simulink model "AFC1_F_trainscg_15_15_15_controller_ep_1000_Nor_20250518"  (R2021a)
settings: Solver=VariableStepAuto  StartTime=0.0  StopTime=10.0  RelTol=1e-3
libraries: neural x50
(part 2 of 2)

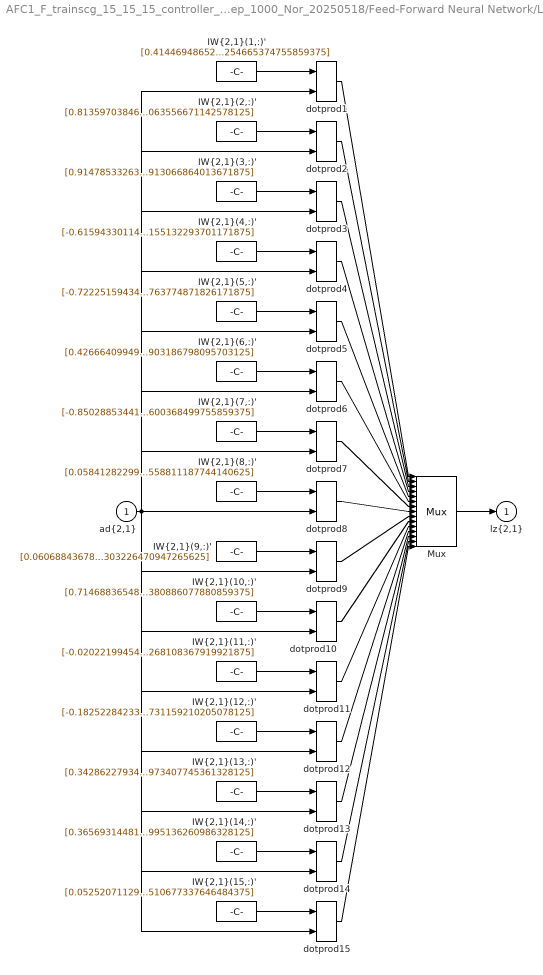
== system AFC1_F_trainscg_15_15_15_controller_ep_1000_Nor_20250518/Feed-Forward Neural Network/Layer 2/LW{2,1} ==
  "ad{2,1}" : Inport  PortDimensions=15
      mask Display: e = 0.06;c1 = [120 230 180]/255;c2 = ([120 230 180]+0)/(256+128);c3 = ([120 230 180]+128)/(256+128);patch([0 1 1 0],[0 0 1 1],c1);patch([0 1 1 1-e 1-e 0+e],[0 0 1 1-e 0+e 0+e],c2);patch([0 0 1 1-e 0+e 0+e],[0 1 1 1-e 1-e 0+e],c3);plot([0 1 1 0 0],[0 0 1 1 0]);
  "IW{2,1}(1,:)'" : Constant  Value=[0.414469486526158281680665140811470337212085723876953125;-0.2259536984836016670907810066637466661632061004638671875;-1.0195501104377717727089702748344279825687408447265625;0.54480850054258167514120714258751831948757171630859375;-0.1760777495828814431799713702275766991078853607177734375;0.5823251328806093862766601887415163218975067138671875;-0.54431412858791627940036050858907401561737060546875;0.5380581706717924017624454791075550019741058349609375;-0.9009348419158775822523921306128613650798797607421875;-0.7521354448038597428904949993011541664600372314453125;0.241917287870616615208518851432017982006072998046875;-0.84101322207548967480050805534119717776775360107421875;-0.64873063937154740177248868349124677479267120361328125;-0.60797567984407063779173086004448123276233673095703125;-0.659413490808771651785491485497914254665374755859375]
      mask Display: e = 0.06;c1 = [120 150 230]/255;c2 = ([120 150 230]+0)/383;c3 = ([120 150 230]+128)/383;patch([0 1 1 0],[0 0 1 1],c1);patch([0 1 1 1-e 1-e 0+e],[0 0 1 1-e 0+e 0+e],c2);patch([0 0 1 1-e 0+e 0+e],[0 1 1 1-e 1-e 0+e],c3);plot([0 1 1 0 0],[0 0 1 1 0]);disp('weights');
  "IW{2,1}(10,:)'" : Constant  Value=[0.7146883654878719571712508695782162249088287353515625;-0.08214663972938236746745843674943898804485797882080078125;0.55044775605694618025864883747999556362628936767578125;0.954649122831302765490590900299139320850372314453125;0.3557796049595560727851761839701794087886810302734375;0.77915393221201278972642967346473596990108489990234375;-0.8330343727947546739187600906006991863250732421875;-0.581189831958130564970588238793425261974334716796875;-0.4362662882391401542037101535242982208728790283203125;-0.588048968935513283184945976245217025279998779296875;0.968796624481943258189176049199886620044708251953125;0.712762216768441536629552501835860311985015869140625;-0.45158776578670067891607686760835349559783935546875;-0.050073148627536485932854048996887286193668842315673828125;-0.1291644265589745044220393310752115212380886077880859375]
      mask Display: e = 0.06;c1 = [120 150 230]/255;c2 = ([120 150 230]+0)/383;c3 = ([120 150 230]+128)/383;patch([0 1 1 0],[0 0 1 1],c1);patch([0 1 1 1-e 1-e 0+e],[0 0 1 1-e 0+e 0+e],c2);patch([0 0 1 1-e 0+e 0+e],[0 1 1 1-e 1-e 0+e],c3);plot([0 1 1 0 0],[0 0 1 1 0]);disp('weights');
  "IW{2,1}(11,:)'" : Constant  Value=[-0.020221994544841991048311768963685608468949794769287109375;0.39058790934535092542745360333356074988842010498046875;-0.267494483371077951261440830421634018421173095703125;0.008683861322354761991260119202706846408545970916748046875;-0.03148972773896197008269837169791571795940399169921875;0.2116872775745909651678999807700165547430515289306640625;0.25191957034316647678906520013697445392608642578125;0.1045826830775500315695580866304226219654083251953125;0.07719335609068078696282100281678140163421630859375;0.8958662425863372913426019295002333819866180419921875;0.7178776333677323595594543803599663078784942626953125;0.0823128711607351848389413362383493222296237945556640625;-0.1821172769517398759564485999362659640610218048095703125;0.784913646248323715326478122733533382415771484375;-1.033094077922761311327803923632018268108367919921875]
      mask Display: e = 0.06;c1 = [120 150 230]/255;c2 = ([120 150 230]+0)/383;c3 = ([120 150 230]+128)/383;patch([0 1 1 0],[0 0 1 1],c1);patch([0 1 1 1-e 1-e 0+e],[0 0 1 1-e 0+e 0+e],c2);patch([0 0 1 1-e 0+e 0+e],[0 1 1 1-e 1-e 0+e],c3);plot([0 1 1 0 0],[0 0 1 1 0]);disp('weights');
  "IW{2,1}(12,:)'" : Constant  Value=[-0.1825228423300189195543907771934755146503448486328125;-0.2116393226556184392617154799154377542436122894287109375;0.61085605728163583361123301074258051812648773193359375;0.7443810798191494715325688957818783819675445556640625;-0.62247861816263128087456379944342188537120819091796875;0.965093447760789313605300776544027030467987060546875;0.32188911589468460761054302565753459930419921875;0.25976677012884241690926501178182661533355712890625;0.390326078888663996480090645491145551204681396484375;-0.835857585804548275376646415679715573787689208984375;0.571117978530061076725132807041518390178680419921875;0.7300334446399059373788986704312264919281005859375;-0.06533126904650272959163004315996658988296985626220703125;-0.7992512801152766854784204042516648769378662109375;0.77556135590495778320274666839395649731159210205078125]
      mask Display: e = 0.06;c1 = [120 150 230]/255;c2 = ([120 150 230]+0)/383;c3 = ([120 150 230]+128)/383;patch([0 1 1 0],[0 0 1 1],c1);patch([0 1 1 1-e 1-e 0+e],[0 0 1 1-e 0+e 0+e],c2);patch([0 0 1 1-e 0+e 0+e],[0 1 1 1-e 1-e 0+e],c3);plot([0 1 1 0 0],[0 0 1 1 0]);disp('weights');
  "IW{2,1}(13,:)'" : Constant  Value=[0.342862279348052023664195075980387628078460693359375;0.366831733935956805225941934622824192047119140625;0.5101541980141670595827463330351747572422027587890625;0.1760521106169949945297048543579876422882080078125;-0.0099883500195583341252358877682127058506011962890625;0.0553601386768847181230057685752399265766143798828125;0.459503710634442175120284446165896952152252197265625;-0.9360179684748661799176261411048471927642822265625;-0.0017679730348210132007125139352865517139434814453125;-0.7885811468365571119676360467565245926380157470703125;0.0267548371751498148540804322692565619945526123046875;-0.3042416113454777804037121313740499317646026611328125;0.5279141569839131964414491449133493006229400634765625;0.4910921474034346534409678497468121349811553955078125;-0.606683617264736074758957329322583973407745361328125]
      mask Display: e = 0.06;c1 = [120 150 230]/255;c2 = ([120 150 230]+0)/383;c3 = ([120 150 230]+128)/383;patch([0 1 1 0],[0 0 1 1],c1);patch([0 1 1 1-e 1-e 0+e],[0 0 1 1-e 0+e 0+e],c2);patch([0 0 1 1-e 0+e 0+e],[0 1 1 1-e 1-e 0+e],c3);plot([0 1 1 0 0],[0 0 1 1 0]);disp('weights');
  "IW{2,1}(14,:)'" : Constant  Value=[0.36569314481354375789834421084378845989704132080078125;0.463132816817762360539489918664912693202495574951171875;-0.307263751603320367511429367368691600859165191650390625;-0.6367346347823830132739431064692325890064239501953125;-0.72715071881299753187022361089475452899932861328125;0.10794316621904233299833464343464584089815616607666015625;0.78150423265064450362160641816444694995880126953125;0.2294268382342810053131643144297413527965545654296875;0.071602111502226506445367704145610332489013671875;-0.7159177561920035959275310233351774513721466064453125;-0.644795078988269931841159632313065230846405029296875;-0.2246800037110795733585888456218526698648929595947265625;0.6264676586349986475710238664760254323482513427734375;0.491901981953333178321230434448807500302791595458984375;-0.8295669794164439725392412583460099995136260986328125]
      mask Display: e = 0.06;c1 = [120 150 230]/255;c2 = ([120 150 230]+0)/383;c3 = ([120 150 230]+128)/383;patch([0 1 1 0],[0 0 1 1],c1);patch([0 1 1 1-e 1-e 0+e],[0 0 1 1-e 0+e 0+e],c2);patch([0 0 1 1-e 0+e 0+e],[0 1 1 1-e 1-e 0+e],c3);plot([0 1 1 0 0],[0 0 1 1 0]);disp('weights');
  "IW{2,1}(15,:)'" : Constant  Value=[0.05252071129474260302583132897780160419642925262451171875;-0.1330683727143766870160135340483975596725940704345703125;-0.5847519347945955292544795156572945415973663330078125;-0.63886919009627873844436862782458774745464324951171875;-0.8971754527457538319623608913389034569263458251953125;0.54648741890165108969767970847897231578826904296875;0.964606445767212772324228353681974112987518310546875;-0.2751770754538946928136056158109568059444427490234375;-0.10963366940791541281896570581011474132537841796875;-0.667079118247158486809667010675184428691864013671875;-0.2028210065283138074931912342435680329799652099609375;-0.877611894985142360070540235028602182865142822265625;-0.79725683317359485879904923422145657241344451904296875;0.124435927059549644724256722838617861270904541015625;-0.416150764835760911264372907680808566510677337646484375]
      mask Display: e = 0.06;c1 = [120 150 230]/255;c2 = ([120 150 230]+0)/383;c3 = ([120 150 230]+128)/383;patch([0 1 1 0],[0 0 1 1],c1);patch([0 1 1 1-e 1-e 0+e],[0 0 1 1-e 0+e 0+e],c2);patch([0 0 1 1-e 0+e 0+e],[0 1 1 1-e 1-e 0+e],c3);plot([0 1 1 0 0],[0 0 1 1 0]);disp('weights');
  "IW{2,1}(2,:)'" : Constant  Value=[0.81359703846538866667259526366251520812511444091796875;-0.69557176260931818934096781958942301571369171142578125;-0.35735248624277360374179579594056122004985809326171875;0.94837000715828800867512882177834399044513702392578125;0.427155190796831452093584857720998115837574005126953125;0.2002273250899879730724251203355379402637481689453125;-0.003811417607220590753058786503970623016357421875;0.162892975750795532263737186440266668796539306640625;-0.0208600216453564968333012075163424015045166015625;-0.0192854130639636967003980316803790628910064697265625;0.147419529682396355241280616610310971736907958984375;-0.963420188137352528912060734000988304615020751953125;0.327449263835897175223266231114394031465053558349609375;-0.2810892969728204793256054472294636070728302001953125;0.189692708737160764531637369145755656063556671142578125]
      mask Display: e = 0.06;c1 = [120 150 230]/255;c2 = ([120 150 230]+0)/383;c3 = ([120 150 230]+128)/383;patch([0 1 1 0],[0 0 1 1],c1);patch([0 1 1 1-e 1-e 0+e],[0 0 1 1-e 0+e 0+e],c2);patch([0 0 1 1-e 0+e 0+e],[0 1 1 1-e 1-e 0+e],c3);plot([0 1 1 0 0],[0 0 1 1 0]);disp('weights');
  "IW{2,1}(3,:)'" : Constant  Value=[0.9147853326346122582179987148265354335308074951171875;0.063908989507247715433635448789573274552822113037109375;-0.14686911338523411796330719880643300712108612060546875;-0.3143718417331886616494784902897663414478302001953125;0.6604950288199826768931188780697993934154510498046875;0.8262060339228549654677635771804489195346832275390625;0.801704977064009671750000052270479500293731689453125;0.856626124628375951175485170097090303897857666015625;-0.6149792078758504754176783535513095557689666748046875;0.7059963106816324884817959173233248293399810791015625;-0.8958442194282607573541099554859101772308349609375;0.8416257669302342758754775786655955016613006591796875;-0.324913212581908472653680064468062482774257659912109375;-0.88494504628262971035468353875330649316310882568359375;-0.369546823609705199498165484328637830913066864013671875]
      mask Display: e = 0.06;c1 = [120 150 230]/255;c2 = ([120 150 230]+0)/383;c3 = ([120 150 230]+128)/383;patch([0 1 1 0],[0 0 1 1],c1);patch([0 1 1 1-e 1-e 0+e],[0 0 1 1-e 0+e 0+e],c2);patch([0 0 1 1-e 0+e 0+e],[0 1 1 1-e 1-e 0+e],c3);plot([0 1 1 0 0],[0 0 1 1 0]);disp('weights');
  "IW{2,1}(4,:)'" : Constant  Value=[-0.6159433011444501726572298139217309653759002685546875;-0.4757093645443852825138719708775170147418975830078125;-0.4594591531358693803355208729044534265995025634765625;0.34252874090347962265923342783935368061065673828125;0.579926059889061651375641304184682667255401611328125;0.3933344011104551452007171974400989711284637451171875;0.1493224382603752786735640256665647029876708984375;0.1601807315168832790419628508971072733402252197265625;-0.753832504908109601871046834276057779788970947265625;0.7478548117234666836594669803162105381488800048828125;0.862402769216499276438980814418755471706390380859375;-0.3973878708272156057290658281999640166759490966796875;0.7969722756685990727731905280961655080318450927734375;0.0437713473225584959180878286133520305156707763671875;-0.7317541343426352540291190962307155132293701171875]
      mask Display: e = 0.06;c1 = [120 150 230]/255;c2 = ([120 150 230]+0)/383;c3 = ([120 150 230]+128)/383;patch([0 1 1 0],[0 0 1 1],c1);patch([0 1 1 1-e 1-e 0+e],[0 0 1 1-e 0+e 0+e],c2);patch([0 0 1 1-e 0+e 0+e],[0 1 1 1-e 1-e 0+e],c3);plot([0 1 1 0 0],[0 0 1 1 0]);disp('weights');
  "IW{2,1}(5,:)'" : Constant  Value=[-0.7222515943416893957618185595492832362651824951171875;-0.9110918154435230231769082820392213761806488037109375;-0.6058924038090884867102658972726203501224517822265625;-0.122710034826088776327424056944437325000762939453125;-0.3629515092020156874497160970349796116352081298828125;0.165581930351680117752266596653498709201812744140625;0.6903563701080732695203323601162992417812347412109375;-0.96603412332547744512112330994568765163421630859375;-0.5890116581846402965538800344802439212799072265625;-0.45941133541460477118789640371687710285186767578125;0.457323363356542333946208600536920130252838134765625;-0.408932331049287167701322687207721173763275146484375;-0.763689603106578740465693044825457036495208740234375;-0.3283020506461509224749306667945347726345062255859375;-0.574796933282314181923311480204574763774871826171875]
      mask Display: e = 0.06;c1 = [120 150 230]/255;c2 = ([120 150 230]+0)/383;c3 = ([120 150 230]+128)/383;patch([0 1 1 0],[0 0 1 1],c1);patch([0 1 1 1-e 1-e 0+e],[0 0 1 1-e 0+e 0+e],c2);patch([0 0 1 1-e 0+e 0+e],[0 1 1 1-e 1-e 0+e],c3);plot([0 1 1 0 0],[0 0 1 1 0]);disp('weights');
  "IW{2,1}(6,:)'" : Constant  Value=[0.426664099491033510513915416595409624278545379638671875;0.51950692946101872937703092247829772531986236572265625;0.651069854811284098872192771523259580135345458984375;0.69164786927618593370681310261716134846210479736328125;0.06607430057406105117223660272429697215557098388671875;0.6963672847159416701146028572111390531063079833984375;0.47728058399080364182509583770297467708587646484375;-0.7582808578028836787865429869270883500576019287109375;-0.7069701787702202810947937905439175665378570556640625;-0.5830772824973724510755346273072063922882080078125;0.4756833075951802936032208890537731349468231201171875;-0.318427681646871629794759428477846086025238037109375;0.97077568772013778097829117541550658643245697021484375;-0.6490654602349377189085544159752316772937774658203125;0.79632667167869553015435712950420565903186798095703125]
      mask Display: e = 0.06;c1 = [120 150 230]/255;c2 = ([120 150 230]+0)/383;c3 = ([120 150 230]+128)/383;patch([0 1 1 0],[0 0 1 1],c1);patch([0 1 1 1-e 1-e 0+e],[0 0 1 1-e 0+e 0+e],c2);patch([0 0 1 1-e 0+e 0+e],[0 1 1 1-e 1-e 0+e],c3);plot([0 1 1 0 0],[0 0 1 1 0]);disp('weights');
  "IW{2,1}(7,:)'" : Constant  Value=[-0.8502885344150248325689744888222776353359222412109375;-0.458571123622145748743861304319580085575580596923828125;-0.1654671363615191348461763709565275348722934722900390625;0.547400866079011283460431513958610594272613525390625;-0.82167642670026330709021067377761937677860260009765625;0.82270153114165023300330403799307532608509063720703125;0.17197407165295164332974309218116104602813720703125;0.725421437399339286145050209597684442996978759765625;-0.621855651054772362584799338947050273418426513671875;0.1299591414764023067363041263888590037822723388671875;-0.8731909986143635560296161202131770551204681396484375;-0.1103551110521081290993805623656953684985637664794921875;0.07529612114779637987993510250817053020000457763671875;-0.5645611733813964416839326077024452388286590576171875;-0.86764964726549675955169504959485493600368499755859375]
      mask Display: e = 0.06;c1 = [120 150 230]/255;c2 = ([120 150 230]+0)/383;c3 = ([120 150 230]+128)/383;patch([0 1 1 0],[0 0 1 1],c1);patch([0 1 1 1-e 1-e 0+e],[0 0 1 1-e 0+e 0+e],c2);patch([0 0 1 1-e 0+e 0+e],[0 1 1 1-e 1-e 0+e],c3);plot([0 1 1 0 0],[0 0 1 1 0]);disp('weights');
  "IW{2,1}(8,:)'" : Constant  Value=[0.058412822999441664506559135361385415308177471160888671875;-0.16459466748032236527166105588548816740512847900390625;0.8118795596206818121487458483898080885410308837890625;-0.63651614818091906133901147768483497202396392822265625;-0.7401005058275689219016157949226908385753631591796875;0.9993359303938624815799585121567361056804656982421875;-0.5065309480280502096860573146841488778591156005859375;-0.031406977575795025359184364788234233856201171875;-0.9146951781777132861606105507235042750835418701171875;0.2806236503255161718328736242256127297878265380859375;0.720881126076463818463935240288265049457550048828125;0.297085696902822604670291184447705745697021484375;0.419601217287414451906357726329588331282138824462890625;0.80640122343862719045404219286865554749965667724609375;-0.465338052563748549861344372402527369558811187744140625]
      mask Display: e = 0.06;c1 = [120 150 230]/255;c2 = ([120 150 230]+0)/383;c3 = ([120 150 230]+128)/383;patch([0 1 1 0],[0 0 1 1],c1);patch([0 1 1 1-e 1-e 0+e],[0 0 1 1-e 0+e 0+e],c2);patch([0 0 1 1-e 0+e 0+e],[0 1 1 1-e 1-e 0+e],c3);plot([0 1 1 0 0],[0 0 1 1 0]);disp('weights');
  "IW{2,1}(9,:)'" : Constant  Value=[0.0606884367857267736923176926211453974246978759765625;0.3755921702402142958732156330370344221591949462890625;-0.2176340090776733848798585313488729298114776611328125;0.72396095740414434516196706681512296199798583984375;-0.727414902123402651312744637834839522838592529296875;-0.9989552492861104582289044628851115703582763671875;0.3328324346389359700282284393324516713619232177734375;0.6897113491525264095116654061712324619293212890625;0.270395833719764056013445951975882053375244140625;-0.16594209671422799345918974722735583782196044921875;0.8688102379224267313162499704048968851566314697265625;-0.9495436370139274107060600726981647312641143798828125;0.9989832401954092944151852861978113651275634765625;0.35078235467249374579523646389134228229522705078125;-0.892491215582572383624437861726619303226470947265625]
      mask Display: e = 0.06;c1 = [120 150 230]/255;c2 = ([120 150 230]+0)/383;c3 = ([120 150 230]+128)/383;patch([0 1 1 0],[0 0 1 1],c1);patch([0 1 1 1-e 1-e 0+e],[0 0 1 1-e 0+e 0+e],c2);patch([0 0 1 1-e 0+e 0+e],[0 1 1 1-e 1-e 0+e],c3);plot([0 1 1 0 0],[0 0 1 1 0]);disp('weights');
  Mux : Mux  Inputs=15
      mask Display: e = 0.06;c1 = [120 150 230]/255;c2 = ([120 150 230]+0)/383;c3 = ([120 150 230]+128)/383;patch([0 1 1 0],[0 0 1 1],c1);patch([0 1 1 1-e 1-e 0+e],[0 0 1 1-e 0+e 0+e],c2);patch([0 0 1 1-e 0+e 0+e],[0 1 1 1-e 1-e 0+e],c3);plot([0 1 1 0 0],[0 0 1 1 0]);disp('Mux');
  dotprod{1..15} (15 alike) : neural/Weight Functions/dotprod
  "lz{2,1}" : Outport
      mask Display: e = 0.06;c1 = [120 230 180]/255;c2 = ([120 230 180]+0)/(256+128);c3 = ([120 230 180]+128)/(256+128);patch([0 1 1 0],[0 0 1 1],c1);patch([0 1 1 1-e 1-e 0+e],[0 0 1 1-e 0+e 0+e],c2);patch([0 0 1 1-e 0+e 0+e],[0 1 1 1-e 1-e 0+e],c3);plot([0 1 1 0 0],[0 0 1 1 0]);
  wires:
  "IW{2,1}(1,:)'"/1 -> dotprod1/1
  "ad{2,1}"/1 -> dotprod1/2, dotprod2/2, dotprod3/2, dotprod4/2, dotprod5/2, dotprod6/2, dotprod7/2, dotprod8/2, dotprod9/2, dotprod10/2, dotprod11/2, dotprod12/2, dotprod13/2, dotprod14/2, dotprod15/2
  dotprod1/1 -> Mux/1
  "IW{2,1}(2,:)'"/1 -> dotprod2/1
  dotprod2/1 -> Mux/2
  "IW{2,1}(3,:)'"/1 -> dotprod3/1
  dotprod3/1 -> Mux/3
  "IW{2,1}(4,:)'"/1 -> dotprod4/1
  dotprod4/1 -> Mux/4
  "IW{2,1}(5,:)'"/1 -> dotprod5/1
  dotprod5/1 -> Mux/5
  "IW{2,1}(6,:)'"/1 -> dotprod6/1
  dotprod6/1 -> Mux/6
  "IW{2,1}(7,:)'"/1 -> dotprod7/1
  dotprod7/1 -> Mux/7
  "IW{2,1}(8,:)'"/1 -> dotprod8/1
  dotprod8/1 -> Mux/8
  "IW{2,1}(9,:)'"/1 -> dotprod9/1
  dotprod9/1 -> Mux/9
  "IW{2,1}(10,:)'"/1 -> dotprod10/1
  dotprod10/1 -> Mux/10
  "IW{2,1}(11,:)'"/1 -> dotprod11/1
  dotprod11/1 -> Mux/11
  "IW{2,1}(12,:)'"/1 -> dotprod12/1
  dotprod12/1 -> Mux/12
  "IW{2,1}(13,:)'"/1 -> dotprod13/1
  dotprod13/1 -> Mux/13
  "IW{2,1}(14,:)'"/1 -> dotprod14/1
  dotprod14/1 -> Mux/14
  "IW{2,1}(15,:)'"/1 -> dotprod15/1
  dotprod15/1 -> Mux/15
  Mux/1 -> "lz{2,1}"/1

== system AFC1_F_trainscg_15_15_15_controller_ep_1000_Nor_20250518/Feed-Forward Neural Network/Layer 3/Delays 1 ==
  "p{3}" : Inport  PortDimensions=15
      mask Display: e = 0.06;c1 = [120 230 180]/255;c2 = ([120 230 180]+0)/(256+128);c3 = ([120 230 180]+128)/(256+128);patch([0 1 1 0],[0 0 1 1],c1);patch([0 1 1 1-e 1-e 0+e],[0 0 1 1-e 0+e 0+e],c2);patch([0 0 1 1-e 0+e 0+e],[0 1 1 1-e 1-e 0+e],c3);plot([0 1 1 0 0],[0 0 1 1 0]);
  mux : Mux  Inputs=1
      mask Display: e = 0.06;c1 = [120 150 230]/255;c2 = ([120 150 230]+0)/383;c3 = ([120 150 230]+128)/383;patch([0 1 1 0],[0 0 1 1],c1);patch([0 1 1 1-e 1-e 0+e],[0 0 1 1-e 0+e 0+e],c2);patch([0 0 1 1-e 0+e 0+e],[0 1 1 1-e 1-e 0+e],c3);plot([0 1 1 0 0],[0 0 1 1 0]);disp('Mux')
  "pd{3,2}" : Outport
      mask Display: e = 0.06;c1 = [120 230 180]/255;c2 = ([120 230 180]+0)/(256+128);c3 = ([120 230 180]+128)/(256+128);patch([0 1 1 0],[0 0 1 1],c1);patch([0 1 1 1-e 1-e 0+e],[0 0 1 1-e 0+e 0+e],c2);patch([0 0 1 1-e 0+e 0+e],[0 1 1 1-e 1-e 0+e],c3);plot([0 1 1 0 0],[0 0 1 1 0]);
  wires:
  "p{3}"/1 -> mux/1
  mux/1 -> "pd{3,2}"/1

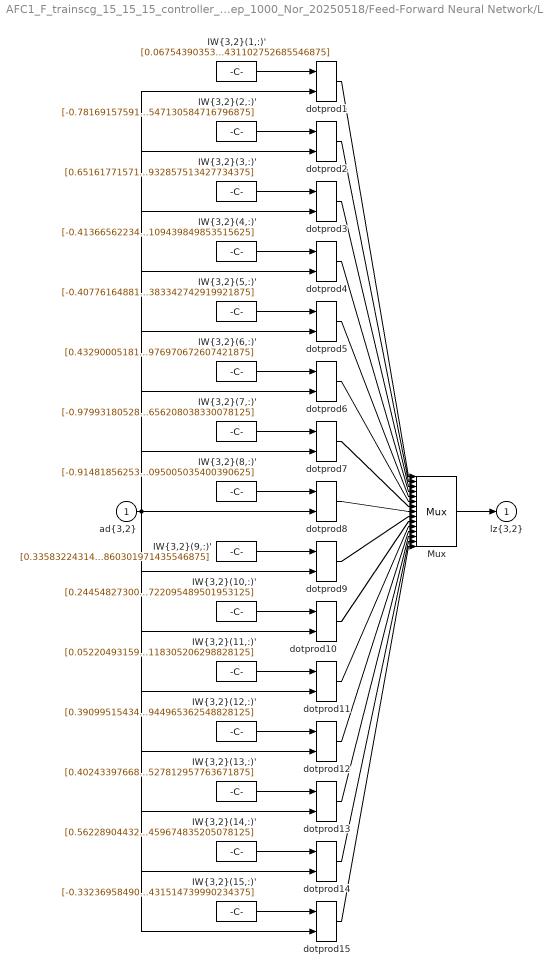
== system AFC1_F_trainscg_15_15_15_controller_ep_1000_Nor_20250518/Feed-Forward Neural Network/Layer 3/LW{3,2} ==
  "ad{3,2}" : Inport  PortDimensions=15
      mask Display: e = 0.06;c1 = [120 230 180]/255;c2 = ([120 230 180]+0)/(256+128);c3 = ([120 230 180]+128)/(256+128);patch([0 1 1 0],[0 0 1 1],c1);patch([0 1 1 1-e 1-e 0+e],[0 0 1 1-e 0+e 0+e],c2);patch([0 0 1 1-e 0+e 0+e],[0 1 1 1-e 1-e 0+e],c3);plot([0 1 1 0 0],[0 0 1 1 0]);
  "IW{3,2}(1,:)'" : Constant  Value=[0.0675439035340004156893201070488430559635162353515625;0.3850639727730376105085952076478861272335052490234375;-0.897336227775257899708094555535353720188140869140625;0.4800646559755552544856982422061264514923095703125;-0.5886509570704803184781894742627628147602081298828125;-0.7754320756879466980393544872640632092952728271484375;-0.0247924491321527273868241536547429859638214111328125;-0.81529532256159686909313677460886538028717041015625;-0.367142001707418064171406513196416199207305908203125;0.9758694699049907939070180873386561870574951171875;-0.2984465102282147785928145822254009544849395751953125;-0.750254482560374302835271009826101362705230712890625;-0.07347884281256167327001094236038625240325927734375;0.61840770258758670507859278586693108081817626953125;0.842194511784394972409018009784631431102752685546875]
      mask Display: e = 0.06;c1 = [120 150 230]/255;c2 = ([120 150 230]+0)/383;c3 = ([120 150 230]+128)/383;patch([0 1 1 0],[0 0 1 1],c1);patch([0 1 1 1-e 1-e 0+e],[0 0 1 1-e 0+e 0+e],c2);patch([0 0 1 1-e 0+e 0+e],[0 1 1 1-e 1-e 0+e],c3);plot([0 1 1 0 0],[0 0 1 1 0]);disp('weights');
  "IW{3,2}(10,:)'" : Constant  Value=[0.2445482730039457985871109713116311468183994293212890625;-0.75693220506058889185396765242330729961395263671875;-0.6966568976520368661198290283209644258022308349609375;0.1958832707677782281052714097313582897186279296875;-0.411867332482743098154287508805282413959503173828125;0.33242139488764232968520673239254392683506011962890625;-0.89186505522761627684502627744222991168498992919921875;-0.69232275049994040916345738878590054810047149658203125;0.8276008215591357242146841599605977535247802734375;0.25326998900797759173286749501130543649196624755859375;-0.1542061110480544561252003177287406288087368011474609375;0.52139336087771626093712029614835046231746673583984375;0.4054046139009506166672736071632243692874908447265625;-0.51410079198184044368957756887539289891719818115234375;0.277510972456713578271347842019167728722095489501953125]
      mask Display: e = 0.06;c1 = [120 150 230]/255;c2 = ([120 150 230]+0)/383;c3 = ([120 150 230]+128)/383;patch([0 1 1 0],[0 0 1 1],c1);patch([0 1 1 1-e 1-e 0+e],[0 0 1 1-e 0+e 0+e],c2);patch([0 0 1 1-e 0+e 0+e],[0 1 1 1-e 1-e 0+e],c3);plot([0 1 1 0 0],[0 0 1 1 0]);disp('weights');
  "IW{3,2}(11,:)'" : Constant  Value=[0.0522049315911223832387122456566430628299713134765625;0.0990802140303959077982653980143368244171142578125;0.2814358459318511140878626974881626665592193603515625;0.5787278872838108600973328066174872219562530517578125;-0.5252539605888415508161415345966815948486328125;-0.780489898553896832567033925442956387996673583984375;-0.3683771233222679075680616733734495937824249267578125;-0.8028118145780045455950357791152782738208770751953125;0.4134304353938611509278189259930513799190521240234375;-0.691260389041455258762880475842393934726715087890625;-0.2807873640555287320097477277158759534358978271484375;0.518654766262192534753694417304359376430511474609375;-0.692819246761199547535170495393685996532440185546875;-0.9589284506836308619170949896215461194515228271484375;0.430425029571680273221545576234348118305206298828125]
      mask Display: e = 0.06;c1 = [120 150 230]/255;c2 = ([120 150 230]+0)/383;c3 = ([120 150 230]+128)/383;patch([0 1 1 0],[0 0 1 1],c1);patch([0 1 1 1-e 1-e 0+e],[0 0 1 1-e 0+e 0+e],c2);patch([0 0 1 1-e 0+e 0+e],[0 1 1 1-e 1-e 0+e],c3);plot([0 1 1 0 0],[0 0 1 1 0]);disp('weights');
  "IW{3,2}(12,:)'" : Constant  Value=[0.390995154348760143303564973393804393708705902099609375;-0.0051261819051731140339800418814775184728205204010009765625;-0.320209101232901638400818455920671112835407257080078125;-0.26469416312424609571962719201110303401947021484375;0.0617445140558567917565824245684780180454254150390625;0.8837869395495001612061969353817403316497802734375;0.56646393646867887472495795009308494627475738525390625;-0.756868460498027584293367908685468137264251708984375;0.1155779335097524285203007821110077202320098876953125;-0.11036106012394315822877643995525431819260120391845703125;0.1170452909097381144487570736600901000201702117919921875;0.57405085820959145248565391739248298108577728271484375;0.90691413977249535349756115465424954891204833984375;0.8954326593311889848081364107201807200908660888671875;0.408097437521362238488364937438745982944965362548828125]
      mask Display: e = 0.06;c1 = [120 150 230]/255;c2 = ([120 150 230]+0)/383;c3 = ([120 150 230]+128)/383;patch([0 1 1 0],[0 0 1 1],c1);patch([0 1 1 1-e 1-e 0+e],[0 0 1 1-e 0+e 0+e],c2);patch([0 0 1 1-e 0+e 0+e],[0 1 1 1-e 1-e 0+e],c3);plot([0 1 1 0 0],[0 0 1 1 0]);disp('weights');
  "IW{3,2}(13,:)'" : Constant  Value=[0.4024339766841695809063139677164144814014434814453125;0.779364213288732177176143522956408560276031494140625;0.261216918251595264788278427658951841294765472412109375;-0.5879442809896107124956188272335566580295562744140625;-0.81700253732117555927061403053812682628631591796875;-0.645761004705822205806953206774778664112091064453125;0.390961489053230859536114394359174184501171112060546875;-0.66878141976656824141400647931732237339019775390625;-0.3731420201268174086095541497343219816684722900390625;-0.73088299229068531825959098569001071155071258544921875;0.476654054502283930361272723530419170856475830078125;0.458682078295435335935081866409745998680591583251953125;0.0817681624829529329900879019987769424915313720703125;0.3070132114268859790939814047305844724178314208984375;-0.17445417493370996009360851530800573527812957763671875]
      mask Display: e = 0.06;c1 = [120 150 230]/255;c2 = ([120 150 230]+0)/383;c3 = ([120 150 230]+128)/383;patch([0 1 1 0],[0 0 1 1],c1);patch([0 1 1 1-e 1-e 0+e],[0 0 1 1-e 0+e 0+e],c2);patch([0 0 1 1-e 0+e 0+e],[0 1 1 1-e 1-e 0+e],c3);plot([0 1 1 0 0],[0 0 1 1 0]);disp('weights');
  "IW{3,2}(14,:)'" : Constant  Value=[0.562289044326892639702464293804951012134552001953125;0.59795177424749501593481681993580423295497894287109375;0.363073558185106060047786513678147457540035247802734375;-0.8266669052089354874368609671364538371562957763671875;-0.189369160238817446639814079389907419681549072265625;-0.52432148433745251470128323489916510879993438720703125;-0.74891920245154486313055031132535077631473541259765625;-0.62153624632020842977198071821476332843303680419921875;-0.6675928741956986822714270601863972842693328857421875;0.377113908643747330895479308310314081609249114990234375;-0.151792258030651161515578451144392602145671844482421875;-0.8581326433859695068662176709040068089962005615234375;0.3594677964209338494327994339982978999614715576171875;0.86472761095639916195665364284650422632694244384765625;-0.21842533575980660476290040605817921459674835205078125]
      mask Display: e = 0.06;c1 = [120 150 230]/255;c2 = ([120 150 230]+0)/383;c3 = ([120 150 230]+128)/383;patch([0 1 1 0],[0 0 1 1],c1);patch([0 1 1 1-e 1-e 0+e],[0 0 1 1-e 0+e 0+e],c2);patch([0 0 1 1-e 0+e 0+e],[0 1 1 1-e 1-e 0+e],c3);plot([0 1 1 0 0],[0 0 1 1 0]);disp('weights');
  "IW{3,2}(15,:)'" : Constant  Value=[-0.332369584909789239635102831016411073505878448486328125;0.43776430620574924290622220723889768123626708984375;0.314407547887482097248579293591319583356380462646484375;0.543867834198214605834209578461013734340667724609375;-0.7903075057684869619833989418111741542816162109375;0.64865034396370446767576822821865789592266082763671875;-0.7658949025320336279065713824820704758167266845703125;-0.280109957530538300485289937569177709519863128662109375;0.244994518559790375178408794454298913478851318359375;0.7613559557717681780530938340234570205211639404296875;-0.139434680302397084883381239706068299710750579833984375;0.341081542930179448802618935587815940380096435546875;-0.926873963903094288951933776843361556529998779296875;-0.73259762910306569505536344877327792346477508544921875;0.47871692694641154730561538599431514739990234375]
      mask Display: e = 0.06;c1 = [120 150 230]/255;c2 = ([120 150 230]+0)/383;c3 = ([120 150 230]+128)/383;patch([0 1 1 0],[0 0 1 1],c1);patch([0 1 1 1-e 1-e 0+e],[0 0 1 1-e 0+e 0+e],c2);patch([0 0 1 1-e 0+e 0+e],[0 1 1 1-e 1-e 0+e],c3);plot([0 1 1 0 0],[0 0 1 1 0]);disp('weights');
  "IW{3,2}(2,:)'" : Constant  Value=[-0.7816915759150828701962154809734784066677093505859375;0.1133396699280251329611246546846814453601837158203125;-0.854229401802047760838831891305744647979736328125;-0.530346170504191416483763532596640288829803466796875;-0.2234567379043965740237354111741296947002410888671875;0.5688557814878254514923128226655535399913787841796875;0.5379165281177382684774102017399854958057403564453125;-0.9843594128613302185470956828794442117214202880859375;-0.564873381154358700229067835607565939426422119140625;-0.6591359538862333611319854753674007952213287353515625;0.3710714174950744403957969552720896899700164794921875;-0.951131967899252028786349910660646855831146240234375;-0.5756735894901312544646998503594659268856048583984375;0.4972377435523942512674011595663614571094512939453125;0.589315770777506298117032201844267547130584716796875]
      mask Display: e = 0.06;c1 = [120 150 230]/255;c2 = ([120 150 230]+0)/383;c3 = ([120 150 230]+128)/383;patch([0 1 1 0],[0 0 1 1],c1);patch([0 1 1 1-e 1-e 0+e],[0 0 1 1-e 0+e 0+e],c2);patch([0 0 1 1-e 0+e 0+e],[0 1 1 1-e 1-e 0+e],c3);plot([0 1 1 0 0],[0 0 1 1 0]);disp('weights');
  "IW{3,2}(3,:)'" : Constant  Value=[0.6516177157111966433689076438895426690578460693359375;-0.20695841483681487460444259340874850749969482421875;-0.8229450806505591575756852762424387037754058837890625;0.4699150833921044156937796287820674479007720947265625;0.103557063914454960951161410775966942310333251953125;-0.416859364186138225960576164652593433856964111328125;-0.2079865095642496886085837104474194347858428955078125;-0.1537812296716669635543439653702080249786376953125;-0.4979163079685278159303152278880588710308074951171875;-0.4844154988559739027920159060158766806125640869140625;-0.4117027324643007801796557032503187656402587890625;-0.4196294697385456462512820507981814444065093994140625;-0.8029625246237832580931126358336769044399261474609375;-0.7596259640258387069167156369076110422611236572265625;0.15478839341329742040898054256103932857513427734375]
      mask Display: e = 0.06;c1 = [120 150 230]/255;c2 = ([120 150 230]+0)/383;c3 = ([120 150 230]+128)/383;patch([0 1 1 0],[0 0 1 1],c1);patch([0 1 1 1-e 1-e 0+e],[0 0 1 1-e 0+e 0+e],c2);patch([0 0 1 1-e 0+e 0+e],[0 1 1 1-e 1-e 0+e],c3);plot([0 1 1 0 0],[0 0 1 1 0]);disp('weights');
  "IW{3,2}(4,:)'" : Constant  Value=[-0.413665622348996731005854599061422049999237060546875;-0.84661605781227466938076986480155028402805328369140625;0.44490693828470406767650047186180017888545989990234375;0.94119705017322896622999905957840383052825927734375;-0.5420934959537999642265049260458908975124359130859375;0.15145076909750476712446243254817090928554534912109375;-0.428628892837826402928413926929351873695850372314453125;0.227153616059499796620002598501741886138916015625;0.785844810571953988898030729615129530429840087890625;-0.233392987233230098098601956735365092754364013671875;0.059238413424801801554497870938575943000614643096923828125;-0.347787464356616948801814714897773228585720062255859375;0.64714894785567711466001128428615629673004150390625;0.108027515504274196356249149175710044801235198974609375;0.029118391415031398550272712100195349194109439849853515625]
      mask Display: e = 0.06;c1 = [120 150 230]/255;c2 = ([120 150 230]+0)/383;c3 = ([120 150 230]+128)/383;patch([0 1 1 0],[0 0 1 1],c1);patch([0 1 1 1-e 1-e 0+e],[0 0 1 1-e 0+e 0+e],c2);patch([0 0 1 1-e 0+e 0+e],[0 1 1 1-e 1-e 0+e],c3);plot([0 1 1 0 0],[0 0 1 1 0]);disp('weights');
  "IW{3,2}(5,:)'" : Constant  Value=[-0.40776164881041321308430269709788262844085693359375;0.55895863107637866473709209458320401608943939208984375;0.873013015130342129310747623094357550144195556640625;0.7338605835038318758734021685086190700531005859375;0.283881240798374623324207277619279921054840087890625;0.92191761577424402585023699430166743695735931396484375;-0.92687473199986480931755750134470872581005096435546875;0.4361612664886107548767313346615992486476898193359375;0.406446449112582097740187236922793090343475341796875;-0.86182937465788655995169165180413983762264251708984375;0.66374200850194553513716755333007313311100006103515625;0.29864298927744992173671789714717306196689605712890625;-0.64998052523584082251772997551597654819488525390625;-0.351906492570844997569423640015884302556514739990234375;-0.492076701060998267234225522770429961383342742919921875]
      mask Display: e = 0.06;c1 = [120 150 230]/255;c2 = ([120 150 230]+0)/383;c3 = ([120 150 230]+128)/383;patch([0 1 1 0],[0 0 1 1],c1);patch([0 1 1 1-e 1-e 0+e],[0 0 1 1-e 0+e 0+e],c2);patch([0 0 1 1-e 0+e 0+e],[0 1 1 1-e 1-e 0+e],c3);plot([0 1 1 0 0],[0 0 1 1 0]);disp('weights');
  "IW{3,2}(6,:)'" : Constant  Value=[0.432900051812038999532461502894875593483448028564453125;-0.304990602924346487778706205062917433679103851318359375;0.267629504596382072900695447970065288245677947998046875;-0.8275309402730073315979097969830036163330078125;-0.0310392552036391489167499457835219800472259521484375;-0.166620373893568485268446011104970239102840423583984375;0.36371436700373338535285938633023761212825775146484375;0.0119897734965194353862205645100402762182056903839111328125;0.1114758854387731812352058113901875913143157958984375;0.348722953937315283123865583547740243375301361083984375;0.1938855891952560861479781806337996385991573333740234375;0.9254979747132459078073907221551053225994110107421875;-0.672860180430013610219930342282168567180633544921875;0.13183287802264620491854429928935132920742034912109375;0.603834211794626707359157080645672976970672607421875]
      mask Display: e = 0.06;c1 = [120 150 230]/255;c2 = ([120 150 230]+0)/383;c3 = ([120 150 230]+128)/383;patch([0 1 1 0],[0 0 1 1],c1);patch([0 1 1 1-e 1-e 0+e],[0 0 1 1-e 0+e 0+e],c2);patch([0 0 1 1-e 0+e 0+e],[0 1 1 1-e 1-e 0+e],c3);plot([0 1 1 0 0],[0 0 1 1 0]);disp('weights');
  "IW{3,2}(7,:)'" : Constant  Value=[-0.97993180528403678319904201998724602162837982177734375;0.2157298051447411879610882579072494991123676300048828125;-0.88549780320721094284408536623232066631317138671875;-0.2671267673616022353400012434576638042926788330078125;-0.6963089497674668226778749158256687223911285400390625;0.294025841296037648842087719458504579961299896240234375;-0.1408710836412364331149404961252002976834774017333984375;-0.77078157856681117632291488916962407529354095458984375;-0.631132664484693517437108312151394784450531005859375;-0.397808567509403798734268775660893879830837249755859375;-0.3132090580302164806170139854657463729381561279296875;0.76279062109329387464384808481554500758647918701171875;0.3319744328222211660062157534412108361721038818359375;-0.20207025700912983889878660193062387406826019287109375;-0.52979250742042005573040341914747841656208038330078125]
      mask Display: e = 0.06;c1 = [120 150 230]/255;c2 = ([120 150 230]+0)/383;c3 = ([120 150 230]+128)/383;patch([0 1 1 0],[0 0 1 1],c1);patch([0 1 1 1-e 1-e 0+e],[0 0 1 1-e 0+e 0+e],c2);patch([0 0 1 1-e 0+e 0+e],[0 1 1 1-e 1-e 0+e],c3);plot([0 1 1 0 0],[0 0 1 1 0]);disp('weights');
  "IW{3,2}(8,:)'" : Constant  Value=[-0.91481856253907023468485704142949543893337249755859375;0.48633601683667093684704241240979172289371490478515625;0.4155599706164443407629960347549058496952056884765625;-0.2616023913399636580123797102714888751506805419921875;0.5638639331760038064800255597219802439212799072265625;0.5042732563250031940782491801655851304531097412109375;-0.093430268941563754392376495161443017423152923583984375;0.2497661201892895921350401522431639023125171661376953125;-0.5759383149353585196195126627571880817413330078125;0.9529344191299433663999707277980633080005645751953125;-0.401946802992273866106387458785320632159709930419921875;-0.08675758422283842696831612784080789424479007720947265625;0.7887787507084855764816211376455612480640411376953125;-0.162760078699813404146112816306413151323795318603515625;-0.85332616656592785719936955501907505095005035400390625]
      mask Display: e = 0.06;c1 = [120 150 230]/255;c2 = ([120 150 230]+0)/383;c3 = ([120 150 230]+128)/383;patch([0 1 1 0],[0 0 1 1],c1);patch([0 1 1 1-e 1-e 0+e],[0 0 1 1-e 0+e 0+e],c2);patch([0 0 1 1-e 0+e 0+e],[0 1 1 1-e 1-e 0+e],c3);plot([0 1 1 0 0],[0 0 1 1 0]);disp('weights');
  "IW{3,2}(9,:)'" : Constant  Value=[0.3358322431472473557079183592577464878559112548828125;-0.7903735160530007686219278184580616652965545654296875;-0.7792930387153027549373973670299164950847625732421875;0.3700569453232185335167514494969509541988372802734375;-0.7987873552751569850016721829888410866260528564453125;-0.1347153477057989601206600127625279128551483154296875;0.2197143385804321003007544277352280914783477783203125;-0.7470002693413941852185189418378286063671112060546875;-0.8453063837746463971001276149763725697994232177734375;-0.195632029555030673151350129046477377414703369140625;-0.0948149168613519055526239753817208111286163330078125;-0.5190432063358307868128349582548253238201141357421875;0.0331164167025408406885844669886864721775054931640625;-0.63852447949041124530822344240732491016387939453125;0.5346590215531488166078588619711808860301971435546875]
      mask Display: e = 0.06;c1 = [120 150 230]/255;c2 = ([120 150 230]+0)/383;c3 = ([120 150 230]+128)/383;patch([0 1 1 0],[0 0 1 1],c1);patch([0 1 1 1-e 1-e 0+e],[0 0 1 1-e 0+e 0+e],c2);patch([0 0 1 1-e 0+e 0+e],[0 1 1 1-e 1-e 0+e],c3);plot([0 1 1 0 0],[0 0 1 1 0]);disp('weights');
  Mux : Mux  Inputs=15
      mask Display: e = 0.06;c1 = [120 150 230]/255;c2 = ([120 150 230]+0)/383;c3 = ([120 150 230]+128)/383;patch([0 1 1 0],[0 0 1 1],c1);patch([0 1 1 1-e 1-e 0+e],[0 0 1 1-e 0+e 0+e],c2);patch([0 0 1 1-e 0+e 0+e],[0 1 1 1-e 1-e 0+e],c3);plot([0 1 1 0 0],[0 0 1 1 0]);disp('Mux');
  dotprod{1..15} (15 alike) : neural/Weight Functions/dotprod
  "lz{3,2}" : Outport
      mask Display: e = 0.06;c1 = [120 230 180]/255;c2 = ([120 230 180]+0)/(256+128);c3 = ([120 230 180]+128)/(256+128);patch([0 1 1 0],[0 0 1 1],c1);patch([0 1 1 1-e 1-e 0+e],[0 0 1 1-e 0+e 0+e],c2);patch([0 0 1 1-e 0+e 0+e],[0 1 1 1-e 1-e 0+e],c3);plot([0 1 1 0 0],[0 0 1 1 0]);
  wires:
  "IW{3,2}(1,:)'"/1 -> dotprod1/1
  "ad{3,2}"/1 -> dotprod1/2, dotprod2/2, dotprod3/2, dotprod4/2, dotprod5/2, dotprod6/2, dotprod7/2, dotprod8/2, dotprod9/2, dotprod10/2, dotprod11/2, dotprod12/2, dotprod13/2, dotprod14/2, dotprod15/2
  dotprod1/1 -> Mux/1
  "IW{3,2}(2,:)'"/1 -> dotprod2/1
  dotprod2/1 -> Mux/2
  "IW{3,2}(3,:)'"/1 -> dotprod3/1
  dotprod3/1 -> Mux/3
  "IW{3,2}(4,:)'"/1 -> dotprod4/1
  dotprod4/1 -> Mux/4
  "IW{3,2}(5,:)'"/1 -> dotprod5/1
  dotprod5/1 -> Mux/5
  "IW{3,2}(6,:)'"/1 -> dotprod6/1
  dotprod6/1 -> Mux/6
  "IW{3,2}(7,:)'"/1 -> dotprod7/1
  dotprod7/1 -> Mux/7
  "IW{3,2}(8,:)'"/1 -> dotprod8/1
  dotprod8/1 -> Mux/8
  "IW{3,2}(9,:)'"/1 -> dotprod9/1
  dotprod9/1 -> Mux/9
  "IW{3,2}(10,:)'"/1 -> dotprod10/1
  dotprod10/1 -> Mux/10
  "IW{3,2}(11,:)'"/1 -> dotprod11/1
  dotprod11/1 -> Mux/11
  "IW{3,2}(12,:)'"/1 -> dotprod12/1
  dotprod12/1 -> Mux/12
  "IW{3,2}(13,:)'"/1 -> dotprod13/1
  dotprod13/1 -> Mux/13
  "IW{3,2}(14,:)'"/1 -> dotprod14/1
  dotprod14/1 -> Mux/14
  "IW{3,2}(15,:)'"/1 -> dotprod15/1
  dotprod15/1 -> Mux/15
  Mux/1 -> "lz{3,2}"/1

== system AFC1_F_trainscg_15_15_15_controller_ep_1000_Nor_20250518/Feed-Forward Neural Network/Layer 4/Delays 1 ==
  "p{4}" : Inport  PortDimensions=15
      mask Display: e = 0.06;c1 = [120 230 180]/255;c2 = ([120 230 180]+0)/(256+128);c3 = ([120 230 180]+128)/(256+128);patch([0 1 1 0],[0 0 1 1],c1);patch([0 1 1 1-e 1-e 0+e],[0 0 1 1-e 0+e 0+e],c2);patch([0 0 1 1-e 0+e 0+e],[0 1 1 1-e 1-e 0+e],c3);plot([0 1 1 0 0],[0 0 1 1 0]);
  mux : Mux  Inputs=1
      mask Display: e = 0.06;c1 = [120 150 230]/255;c2 = ([120 150 230]+0)/383;c3 = ([120 150 230]+128)/383;patch([0 1 1 0],[0 0 1 1],c1);patch([0 1 1 1-e 1-e 0+e],[0 0 1 1-e 0+e 0+e],c2);patch([0 0 1 1-e 0+e 0+e],[0 1 1 1-e 1-e 0+e],c3);plot([0 1 1 0 0],[0 0 1 1 0]);disp('Mux')
  "pd{4,3}" : Outport
      mask Display: e = 0.06;c1 = [120 230 180]/255;c2 = ([120 230 180]+0)/(256+128);c3 = ([120 230 180]+128)/(256+128);patch([0 1 1 0],[0 0 1 1],c1);patch([0 1 1 1-e 1-e 0+e],[0 0 1 1-e 0+e 0+e],c2);patch([0 0 1 1-e 0+e 0+e],[0 1 1 1-e 1-e 0+e],c3);plot([0 1 1 0 0],[0 0 1 1 0]);
  wires:
  "p{4}"/1 -> mux/1
  mux/1 -> "pd{4,3}"/1

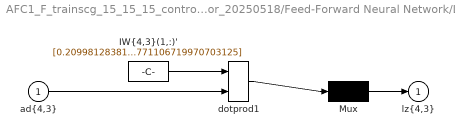
== system AFC1_F_trainscg_15_15_15_controller_ep_1000_Nor_20250518/Feed-Forward Neural Network/Layer 4/LW{4,3} ==
  "ad{4,3}" : Inport  PortDimensions=15
      mask Display: e = 0.06;c1 = [120 230 180]/255;c2 = ([120 230 180]+0)/(256+128);c3 = ([120 230 180]+128)/(256+128);patch([0 1 1 0],[0 0 1 1],c1);patch([0 1 1 1-e 1-e 0+e],[0 0 1 1-e 0+e 0+e],c2);patch([0 0 1 1-e 0+e 0+e],[0 1 1 1-e 1-e 0+e],c3);plot([0 1 1 0 0],[0 0 1 1 0]);
  "IW{4,3}(1,:)'" : Constant  Value=[0.20998128381651870455470998422242701053619384765625;-0.2255091370337301004411756366607733070850372314453125;-0.7156256814189918546986746150651015341281890869140625;-0.76611743866967552119007223154767416417598724365234375;0.1324710757732594779145784968932275660336017608642578125;-0.62747605654755667092814519492094404995441436767578125;0.357849961214182721302989875766797922551631927490234375;-0.056999592006650785791510571698381681926548480987548828125;0.683120174936412194455215285415761172771453857421875;0.37362916393967549044674569813651032745838165283203125;0.142051745648757776763204674352891743183135986328125;-0.81141351895158086993120605256990529596805572509765625;0.91209023535646738256588150761672295629978179931640625;-0.444703553668884532523719599339528940618038177490234375;0.81746490272565008883276505002868361771106719970703125]
      mask Display: e = 0.06;c1 = [120 150 230]/255;c2 = ([120 150 230]+0)/383;c3 = ([120 150 230]+128)/383;patch([0 1 1 0],[0 0 1 1],c1);patch([0 1 1 1-e 1-e 0+e],[0 0 1 1-e 0+e 0+e],c2);patch([0 0 1 1-e 0+e 0+e],[0 1 1 1-e 1-e 0+e],c3);plot([0 1 1 0 0],[0 0 1 1 0]);disp('weights');
  Mux : Mux  Inputs=1
      mask Display: e = 0.06;c1 = [120 150 230]/255;c2 = ([120 150 230]+0)/383;c3 = ([120 150 230]+128)/383;patch([0 1 1 0],[0 0 1 1],c1);patch([0 1 1 1-e 1-e 0+e],[0 0 1 1-e 0+e 0+e],c2);patch([0 0 1 1-e 0+e 0+e],[0 1 1 1-e 1-e 0+e],c3);plot([0 1 1 0 0],[0 0 1 1 0]);disp('Mux');
  dotprod1 : neural/Weight Functions/dotprod
  "lz{4,3}" : Outport
      mask Display: e = 0.06;c1 = [120 230 180]/255;c2 = ([120 230 180]+0)/(256+128);c3 = ([120 230 180]+128)/(256+128);patch([0 1 1 0],[0 0 1 1],c1);patch([0 1 1 1-e 1-e 0+e],[0 0 1 1-e 0+e 0+e],c2);patch([0 0 1 1-e 0+e 0+e],[0 1 1 1-e 1-e 0+e],c3);plot([0 1 1 0 0],[0 0 1 1 0]);
  wires:
  "IW{4,3}(1,:)'"/1 -> dotprod1/1
  "ad{4,3}"/1 -> dotprod1/2
  dotprod1/1 -> Mux/1
  Mux/1 -> "lz{4,3}"/1
